simulink model "ex6_i2c"  (Simulink 7.6)
settings: Solver=FixedStepDiscrete  SolverMode=SingleTasking  StartTime=0.0  StopTime=10.0  FixedStep=0.001  RelTol=1e-3
libraries: dsPICdrivers x6
settings Model: Creator=Lior  LastModifiedBy=Lior
settings OptimizationCC: OptimizeModelRefInitCode=on  LifeSpan=1
settings HardwareCC: ProdBitPerInt=16  ProdBitPerPointer=16  ProdEndianess=LittleEndian  ProdWordSize=16  ProdHWDeviceType=16-bit Generic
settings RTWCC: SystemTargetFile=dspic.tlc  GenCodeOnly=on  MakeCommand=make_CreateMPLAB  TemplateMakefile=dspic_pic30_gcc.tmf  PostCodeGenCommand=dsPIC_Compile()  Description=Embedded Target for Microchip dsPIC (real-time)  ProcessScript=dspic_make_rtw_hook
settings CodeAppCC: IgnoreCustomStorageClasses=off
settings STFCustomTargetCC: IncludeMdlTerminateFcn=off  CombineOutputUpdateFcns=on  SuppressErrorStatus=on  ERTCustomFileBanners=on  SupportContinuousTime=off  SupportNonInlinedSFcns=off  SystemTargetFile=dspic.tlc
settings ERTTargetCC: MultiwordLength=2048  ParMdlRefBuildCompliant=off  CompOptLevelCompliant=off  IncludeMdlTerminateFcn=off  SuppressErrorStatus=on  ERTFirstTimeCompliant=off  ModelStepFunctionPrototypeControlCompliant=off  CPPClassGenCompliant=off  ExtModeMexFile=ext_serial_win32_comm  InlinedParameterPlacement=NonHierarchical  ERTSrcFileBannerTemplate=dsPIC_code_template.cgt  ERTHdrFileBannerTemplate=dsPIC_code_template.cgt  ERTDataSrcFileTemplate=dsPIC_code_template.cgt  ERTDataHdrFileTemplate=dsPIC_code_template.cgt  ERTCustomFileTemplate=dsPIC_main.tlc  ConvertIfToSwitch=off
settings CustomProperty: DataType=string  Value=C:\PROGRA~1\MATLAB\R2010b\bin\win64\gmake

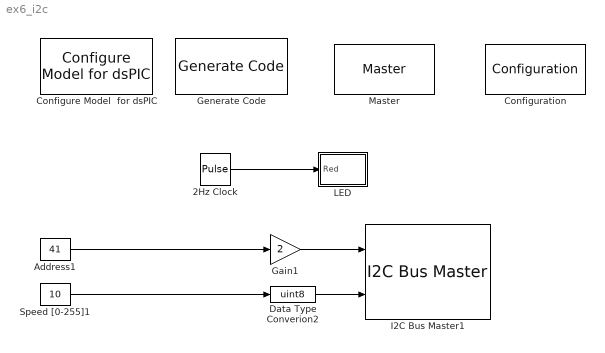
== system ex6_i2c ==
  2Hz Clock : DiscretePulseGenerator  PulseType=Time based  Period=1  PulseWidth=50
  Address1 : Constant  Value=41  OutDataTypeStr=uint8
  Configuration : dsPICdrivers/Configuration  SystemSampleTime=-1  double64=off
  Configure Model  for dsPIC : dsPICdrivers/Simulink Configuration/Configure Model  for dsPIC
  Data Type Converion2 : DataTypeConversion  OutDataTypeStr=uint8
  Gain1 : Gain  Gain=2  OutDataTypeStr=uint8
  Generate Code : dsPICdrivers/Simulink Configuration/Generate Code
  I2C Bus Master1 : dsPICdrivers/BUS I2C/I2C Bus Master  Tag=dsPIC_I2C_Master  NumI2C=1  AltI2C=off  Sequence='S A W P'  InitializeOnceOnly=When I2C bus is enable (if Enable I2C is checked)  Enable=on  WaitAfterEnable=4  Disable=on  AdressNbrBits=7 bits  I2CBusFreq=153  SlewRate=off  SMBUSThreshold=off  OutputErrorFlag=off  SampleTime=0.01  OrderingInOutPopup=None  Info=Fscl = 16 KHz
  LED : Subsystem
  Master : dsPICdrivers/Master  Tag=dsPIC_MASTER  Priority=1  TimeStepType=Timer1  picType=30f4011  fcy=2500000  Quartz_33f=5e6  PLLActive_33f=off  fcyDesired_33f=0  tmr1="[1  2499  0]"  tmr1Info="Time Step : 0.001  ;   Error : 0%  PR1=2499"  tmr2345="[0  0  0  0]"  tmr2345cfg=[-1 -1 -1 -1]  IOautoConf=on  typePort="[ 0   0   0   0   0   0   0   0   0   0   0   0   0   0   0   0  10   0   0   0   0   0   0   0   0   0   0   0   0   0   0   0   0   0   0   0   0   0   0   0   0   0   0   0   0   0   0   0   0   0   0   0   0   0   0   0   0   0   0   0   0   0   0   0   0   0   0   0   0   0   0   0   0   0   0   0   0   0   0   0   0   0  20  20   0   0   0   0   0   0   0   0   0   0   0   0   0   0   0   0   0   0   0   0   0   0   0   0   0   0   0   0 ]"  TRIS="[ 65535  65534  65535  65535  65535  65535  65535 ]"  ADPCFG=1  MasterBusyPort=None  MasterOverloadPort=None  FOSC=CSW_FSCM_OFF  ClockSwitchMonitor=Both disabled  TempProtection_33f=TEMP_ON  FPBOR=PBOR_OFF  PWRT=PWRT_OFF  MCLR=MCLR_EN  ICD=ICS_PGD1  JTAGEN=JTAGEN_OFF  PowerSave=off  OverrideFcy=off  NewFcy=1e6  PR2345="[65535  65535  65535  65535]"
  Speed [0-255]1 : Constant  Value=10  OutDataTypeStr=uint8
  wires:
  Gain1/1 -> I2C Bus Master1/1
  Data Type Converion2/1 -> I2C Bus Master1/2
  Speed [0-255]1/1 -> Data Type Converion2/1
  2Hz Clock/1 -> LED/1(Red)
  Address1/1 -> Gain1/1

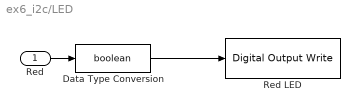
== system ex6_i2c/LED ==
  Red : Inport
  Data Type Conversion : DataTypeConversion  OutDataTypeStr=boolean
  Red LED : dsPICdrivers/Digital I//O/Digital Output Write  Tag=dsPIC_Digital_Output  Priority=5  PORT=B  Pin=[0]  Simultaneous=off  OrderingInOutPopup=None
  wires:
  Data Type Conversion/1 -> Red LED/1
  Red/1 -> Data Type Conversion/1
